simulink model "UPS_Vienna_TNPC"  (R2023b)
settings: Solver=ode45  StartTime=0.0  StopTime=0.5  RelTol=1e-3  EnableMultiTasking=on
libraries: spsSeriesRLCBranchLib x6, spsMosfetLib x6, spsCurrentMeasurementLib x4, spsVoltageMeasurementLib x4, spsDiodeLib x4, simulink x3, powerlib_extras x2, spsIGBTDiodeLib x2, spsTHDLib x2, spsACVoltageSourceLib x1, spsMeanLib x1, slpidlib x1
settings Model: SimulationMode=accelerator  Creator=bzz  LastModifiedBy=Qu
settings SolverCC: ZeroCrossAlgorithm=Adaptive  AlgebraicLoopSolver=TrustRegion
settings DataIOCC: LimitDataPoints=on  ReturnWorkspaceOutputs=off
settings OptimizationCC: LifeSpan=inf
settings DebuggingCC: AlgebraicLoopMsg=none  IgnoredZcDiagnostic=none  UnconnectedInputMsg=warning  UnconnectedOutputMsg=warning  UnconnectedLineMsg=warning  AllowSymbolicDim=off  SFUnexpectedBacktrackingDiag=warning  SFNoUnconditionalDefaultTransitionDiag=warning  ArithmeticOperatorsInVariantConditions=warning
settings ModelReferenceCC: EnableRefExpFcnMdlSchedulingChecks=on  PropagateSignalLabelsOutOfModel=off
settings SFSimCC: SimUseLocalCustomCode=off  CustomCodeUndefinedFunction=UseInterfaceOnly
settings RTWCC: RTWUseLocalCustomCode=off  DLArmComputeVersion=19.05
settings CodeAppCC: StateflowObjectComments=on
settings GRTTargetCC: TargetLangStandard=C89/C90 (ANSI)
settings ConfigComp: CovMetricSettings=dw  CovSaveCumulativeToWorkspaceVar=on  CovSaveSingleToWorkspaceVar=on  CovExternalEMLEnable=off
settings SimscapeCC: SimscapeNormalizeSystem=off

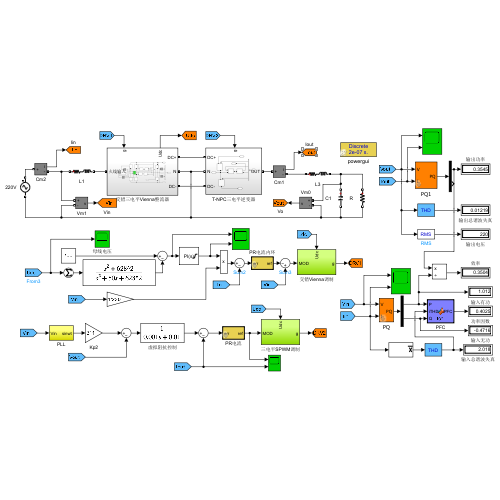
[thumbnail: Simulink's stored preview of the top-level diagram]
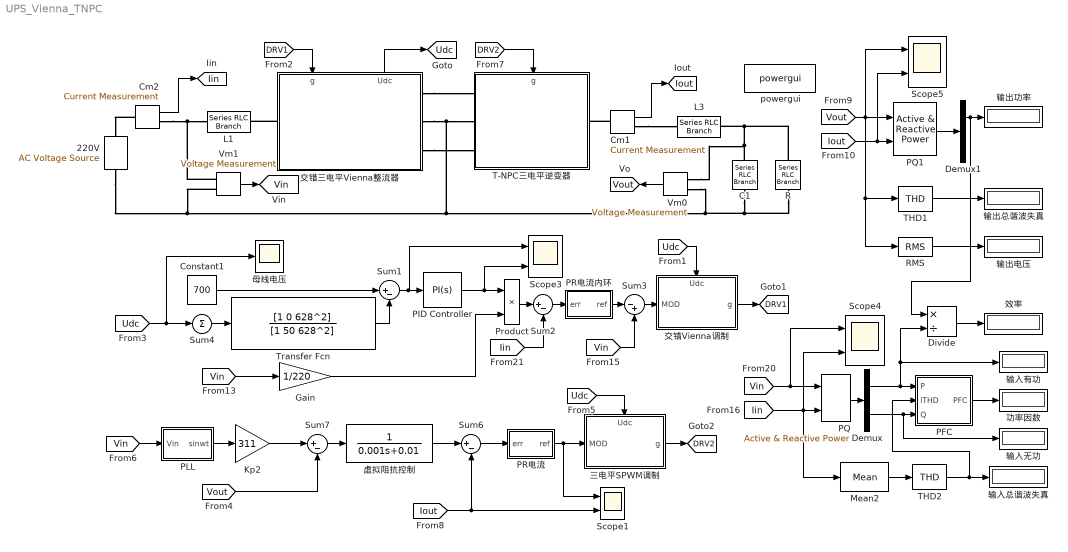
== system UPS_Vienna_TNPC ==
  220V : spsACVoltageSourceLib/AC Voltage Source  Amplitude=225*1.4  Phase=0  Frequency=50  SampleTime=0  Measurements=None  BusType=swing  Pref=10e3  Qref=0  Qmin=-inf  Qmax=+inf
  C1 : spsSeriesRLCBranchLib/Series RLC Branch  LConnTagsString=__new0  RConnTagsString=__new0  BranchType=C  Resistance=0.1  Inductance=0  SetiL0=off  InitialCurrent=0  Capacitance=6e-6  Setx0=off  InitialVoltage=310  Measurements=None
  Cm1 : spsCurrentMeasurementLib/Current Measurement  PhasorSimulation=off  OutputType=Complex  PSBequivalent=0
  Cm2 : spsCurrentMeasurementLib/Current Measurement  PhasorSimulation=off  OutputType=Complex  PSBequivalent=0
  Constant1 : Constant  Value=700
  Demux : Demux  Outputs=2
  Demux1 : Demux  Outputs=2
  Divide : Product  Inputs=*/
  Gain : Gain  Gain=1/220
  Kp2 : Gain  Gain=311
  L1 : spsSeriesRLCBranchLib/Series RLC Branch  LConnTagsString=__new0  RConnTagsString=__new0  BranchType=RL  Resistance=0.01  Inductance=3e-4  SetiL0=off  InitialCurrent=0  Capacitance=inf  Setx0=off  InitialVoltage=0  Measurements=None
  L3 : spsSeriesRLCBranchLib/Series RLC Branch  LConnTagsString=__new0  RConnTagsString=__new0  BranchType=RL  Resistance=0.01  Inductance=6e-4  SetiL0=off  InitialCurrent=0  Capacitance=inf  Setx0=off  InitialVoltage=0  Measurements=None
  Mean2 : spsMeanLib/Mean  Freq=10000  Vinit=0  Ts=0
  PFC : MATLAB Function  TreatAsAtomicUnit=on
  PID Controller : slpidlib/PID Controller  Controller=PI  Form=Parallel  TimeDomain=Continuous-time  UseExternalTs=off  SampleTime=-1  IntegratorMethod=Forward Euler  FilterMethod=Forward Euler  ControllerParametersSource=internal  P=0.2  I=4  UseKiTs=off  D=0.001  N=100  UseFilter=on  TunerSelectOption=Transfer Function Based (PID Tuner App)  InitialConditionSource=internal  InitialConditionForIntegrator=0  InitialConditionForFilter=0  DifferentiatorICPrevScaledInput=0  ExternalReset=none  TrackingMode=off  Kt=1  LimitOutput=on  SatLimitsSource=internal  UpperSaturationLimit=200  LowerSaturationLimit=-200  LinearizeAsGain=on  AntiWindupMode=clamping  Kb=1  LimitIntegrator=off  UpperIntegratorSaturationLimit=inf  LowerIntegratorSaturationLimit=-inf  POutMin=[]  POutMax=[]  IOutMin=[]  IOutMax=[]  DOutMin=[]  DOutMax=[]  NOutMin=[]  NOutMax=[]  SumOutMin=[]  SumOutMax=[]  SaturationOutMin=[]  SaturationOutMax=[]  PParamMin=[]  PParamMax=[]  IParamMin=[]  IParamMax=[]  DParamMin=[]  DParamMax=[]  NParamMin=[]  NParamMax=[]  KbParamMin=[]  KbParamMax=[]  KtParamMin=[]  KtParamMax=[]  KbOutMin=[]  KbOutMax=[]  KtOutMin=[]  KtOutMax=[]  IntegratorOutMin=[]  IntegratorOutMax=[]  FilterOutMin=[]  FilterOutMax=[]  SumI1OutMin=[]  SumI1OutMax=[]  SumI2OutMin=[]  SumI2OutMax=[]  SumI3OutMin=[]  SumI3OutMax=[]  SumI4OutMin=[]  SumI4OutMax=[]  SumDOutMin=[]  SumDOutMax=[]  DifferentiatorOutMin=[]  DifferentiatorOutMax=[]  FilterDiffOutCoefMin=[]  FilterDiffOutCoefMax=[]  ReciprocalOutMin=[]  ReciprocalOutMax=[]  SumDenOutMin=[]  SumDenOutMax=[]  SumNumOutMin=[]  SumNumOutMax=[]  DivideOutMin=[]  DivideOutMax=[]  UdiffTsProdOutMin=[]  UdiffTsProdOutMax=[]  NTsProdOutMin=[]  NTsProdOutMax=[]  UintegralTsProdOutMin=[]  UintegralTsProdOutMax=[]  UngainTsProdOutMin=[]  UngainTsProdOutMax=[]  ClampingZeroOutDataTypeStr=Inherit: Inherit via back propagation  ClampingZeroOutMin=[]  ClampingZeroOutMax=[]  FilterDenConstantOutDataTypeStr=Inherit: Inherit via back propagation  FilterDenConstantOutMin=[]  FilterDenConstantOutMax=[]  PCopyOutDataTypeStr=Inherit: Inherit via back propagation  PCopyOutMin=[]  PCopyOutMax=[]  NCopyOutDataTypeStr=Inherit: Inherit via back propagation  NCopyOutMin=[]  NCopyOutMax=[]  IntegratorContinuousStateAttributes=''  IntegratorStateMustResolveToSignalObject=off  IntegratorRTWStateStorageClass=Auto  FilterContinuousStateAttributes=''  FilterStateMustResolveToSignalObject=off  FilterRTWStateStorageClass=Auto  ParallelPVariant=InternalParameters  IdealPVariant=Disabled  IVariant=InternalParameters  DVariant=Disabled  IntegratorVariant=Continuous  SatVariant=Enabled  AWVariant=ContClampingParallel  PCopyVariant=Disabled  TRVariant=Disabled  FdbkBlocksVariant=Forward  IdealPFdbkVariant=Disabled  SatFdbkVariant=Disabled  DerivativeFilterVariant=Disabled  NVariant=Disabled  NCopyVariant=Disabled_SignalSpec  FilterICVariant=Disabled  IntegratorICVariant=InternalICs  ExternalResetVariant=Disabled  TRSumVariant=Passthrough  SumFdbkVariant=Disabled  SumVariant=Sum_PI  TsampFilterVariant=InternalTs  TsampNgainVariant=Passthrough  TsampIntegralVariant=Disabled_SignalSpec  ExternalSaturationOutDataTypeStr=Inherit: Same as second input
  PLL : Subsystem
  PQ : powerlib_extras/Measurements/Active & Reactive Power  f1=50
  PQ1 : powerlib_extras/Measurements/Active & Reactive Power  f1=50
  PR电流 : Subsystem  TreatAsAtomicUnit=on  mask{Kp=2, Kr=300, Wc=5, Upper=1000, Lower=-1000}
  PR电流内环 : Subsystem  TreatAsAtomicUnit=on  mask{Kp=6, Kr=100, Wc=5, Upper=310, Lower=-310}
  Product : Product
  R : spsSeriesRLCBranchLib/Series RLC Branch  LConnTagsString=__new0  RConnTagsString=__new0  BranchType=R  Resistance=15  Inductance=0  SetiL0=off  InitialCurrent=0  Capacitance=1e-5  Setx0=off  InitialVoltage=310  Measurements=None
  RMS : spsRMSLib/RMS  TrueRMS=on  Freq=50  RMSInit=200  Ts=0
  Scope{1,3..5} (4 alike) : Scope  NumInputPorts=2
  Sum{1..2,6..7} (4 alike) : Sum  Inputs=|+-
  Sum3 : Sum  Inputs=|-+
  Sum4 : Sum  Inputs=+
  T-NPC三电平逆变器 : Subsystem
      settings: PortSchema="{\"entries\":[{\"content\":{\"sides\":[{\"content\":{\"connectorIds\":[\"LConn1\",\"LConn2\",\"LConn3\"]},\"type\":\"ConnectorPlacement.EquallySpacedRectSide\",\"uuid\":\"7489be24-fb05-4397-99c4-0805e15884ae\"},{\"content\":{\"connectorIds\":[\"RConn1\"],\"side\":\"RIGHT\"},\"type\":\"ConnectorPlacement.EquallySpacedRectSide\",\"uuid\":\"654e1801-31b1-421a-885f-2131c51cad8d\"},{\"content\":{\"connectorIds\":[\"In1\"],\"side\":\"TOP\"},\"type\":\"ConnectorPlacement.EquallySpacedRectSide\",\"uuid\":\"fb480e4b-a2b2-44a5-99b2-e83f2782ffff\"},{\"content\":{\"side\":\"BOTTOM\"},\"type\":\"ConnectorPlacement.EquallySpacedRectSide\",\"uuid\":\"4af6c17e-9b76-400a-bd3e-3ab3838d4ab0\"}]},\"type\":\"ConnectorPlacement.EquallySpacedConnector\",\"uuid\":\"da460d4a-b9c7-40d8-ac01-f49018117654\"}],\"packageUris\":[\"http://schema.mathworks.com/mf0/Connector/R2020b\"],\"version\":\"1.0\"}"
  THD1 : spsTHDLib/THD  Freq=50  Ts=0
  THD2 : spsTHDLib/THD  Freq=50  Ts=0
  Transfer Fcn : TransferFcn  Numerator=[1 0 628^2]  Denominator=[1 50 628^2]
  Vm0 : spsVoltageMeasurementLib/Voltage Measurement  PhasorSimulation=off  OutputType=Complex  PSBequivalent=0
  Vm1 : spsVoltageMeasurementLib/Voltage Measurement  PhasorSimulation=off  OutputType=Complex  PSBequivalent=0
  powergui : spspowerguiLib/powergui  SimulationMode=Discrete  SampleTime=2e-7  frequency=60  Iterations=50  frequencyindice=0  Pbase=100e6  ErrMax=1e-4  UnitsV=kV  UnitsW=MW  buscounter=0  FunctionMessages=off  echomessages=off  EnableUseOfTLC=off  CurrentSourceSwitches=off  DisableSnubberDevices=off  DisableRonSwitches=off  DisableVfSwitches=off  DisplayEquations=off  AutomaticDiscreteSolvers=off  SolverType=Tustin/Backward Euler (TBE)  Interpol=off  ExternalGateDelay=off  methode=off  Ts=0  x0status=blocks  SPID=off  SwTol=0  HookPort=off  NonlinearTolerance=1e-4  nMaxIteration=100  ContinueOnMaxIteration=off  RestoreLinks=warning  ResistiveCurrentMeasurement=off  Frange=[0:2:500]  Ylog=off  Xlog=on  ShowGrid=off  save=off  variable=ZData  structure=QQQQQ  ZoomFFT=off  StartTime=0.5  cycles=15  DisplayStyle=1  fundamental=50  FreqAxis=off  MaxFrequency=1000  frequencyindicesteady=1  RmsSteady=1  display=off
  三电平SPWM调制 : Subsystem
      settings: PortSchema="{\"entries\":[{\"content\":{\"sides\":[{\"content\":{\"connectorIds\":[\"In1\"]},\"type\":\"ConnectorPlacement.EquallySpacedRectSide\",\"uuid\":\"1b638a2d-5755-4ae9-be2e-6e83381e6ec7\"},{\"content\":{\"connectorIds\":[\"Out1\"],\"side\":\"RIGHT\"},\"type\":\"ConnectorPlacement.EquallySpacedRectSide\",\"uuid\":\"c11d6821-83ca-44ae-8b26-9c21f079c52d\"},{\"content\":{\"connectorIds\":[\"In2\"],\"side\":\"TOP\"},\"type\":\"ConnectorPlacement.EquallySpacedRectSide\",\"uuid\":\"290bd415-8c82-45df-a08c-f8079695ccf4\"}]},\"type\":\"ConnectorPlacement.EquallySpacedConnector\",\"uuid\":\"c88eaf66-3c08-44e5-8886-a76105e28a39\"}],\"packageUris\":[\"http://schema.mathworks.com/mf0/Connector/R2020b\"],\"version\":\"1.0\"}"
  交错Vienna调制 : Subsystem
      settings: PortSchema="{\"entries\":[{\"content\":{\"sides\":[{\"content\":{\"connectorIds\":[\"In1\"]},\"type\":\"ConnectorPlacement.EquallySpacedRectSide\",\"uuid\":\"1b638a2d-5755-4ae9-be2e-6e83381e6ec7\"},{\"content\":{\"connectorIds\":[\"Out1\"],\"side\":\"RIGHT\"},\"type\":\"ConnectorPlacement.EquallySpacedRectSide\",\"uuid\":\"c11d6821-83ca-44ae-8b26-9c21f079c52d\"},{\"content\":{\"connectorIds\":[\"In2\"],\"side\":\"TOP\"},\"type\":\"ConnectorPlacement.EquallySpacedRectSide\",\"uuid\":\"290bd415-8c82-45df-a08c-f8079695ccf4\"}]},\"type\":\"ConnectorPlacement.EquallySpacedConnector\",\"uuid\":\"c88eaf66-3c08-44e5-8886-a76105e28a39\"}],\"packageUris\":[\"http://schema.mathworks.com/mf0/Connector/R2020b\"],\"version\":\"1.0\"}"
  交错三电平Vienna整流器 : Subsystem
      settings: PortSchema="{\"entries\":[{\"content\":{\"sides\":[{\"content\":{\"connectorIds\":[\"LConn1\"]},\"type\":\"ConnectorPlacement.EquallySpacedRectSide\",\"uuid\":\"7489be24-fb05-4397-99c4-0805e15884ae\"},{\"content\":{\"connectorIds\":[\"RConn1\",\"RConn2\",\"RConn3\"],\"side\":\"RIGHT\"},\"type\":\"ConnectorPlacement.EquallySpacedRectSide\",\"uuid\":\"654e1801-31b1-421a-885f-2131c51cad8d\"},{\"content\":{\"connectorIds\":[\"In1\",\"Out1\"],\"side\":\"TOP\"},\"type\":\"ConnectorPlacement.EquallySpacedRectSide\",\"uuid\":\"fb480e4b-a2b2-44a5-99b2-e83f2782ffff\"},{\"content\":{\"side\":\"BOTTOM\"},\"type\":\"ConnectorPlacement.EquallySpacedRectSide\",\"uuid\":\"4af6c17e-9b76-400a-bd3e-3ab3838d4ab0\"}]},\"type\":\"ConnectorPlacement.EquallySpacedConnector\",\"uuid\":\"da460d4a-b9c7-40d8-ac01-f49018117654\"}],\"packageUris\":[\"http://schema.mathworks.com/mf0/Connector/R2020b\"],\"version\":\"1.0\"}"
  功率因数 : Display
  效率 : Display
  母线电压 : Scope
  虚拟阻抗控制 : TransferFcn  Numerator=1  Denominator=[0.001 0.01]
  输入总谐波失真 : Display
  输入无功 : Display
  输入有功 : Display
  输出功率 : Display
  输出总谐波失真 : Display
  输出电压 : Display
  tag scope: DRV1=global, DRV2=global, Iin=global, Iout=global, Udc=global, Vin=global, Vout=global
  wires:
  PQ/1 -> Demux/1
  Demux/2 -> 输入无功/1, PFC/3(Q)
  PFC/1(PFC) -> 功率因数/1
  Demux/1 -> Divide/2, 输入有功/1, PFC/1(P)
  Cm1/1 -> [Iout]
  THD1/1 -> 输出总谐波失真/1
  Sum1/1 -> Scope3/1, PID Controller/1
  [Vin] -> PQ/1, Scope4/1
  Mean2/1 -> THD2/1
  THD2/1 -> 输入总谐波失真/1, PFC/2(iTHD)
  PR电流内环/1(ref) -> Sum3/1
  [Iin] -> Sum2/2
  Sum2/1 -> PR电流内环/1(err)
  Product/1 -> Sum2/1
  PID Controller/1 -> Product/1, Scope3/2
  交错Vienna调制/1(g) -> [DRV1]
  Constant1/1 -> Sum1/1
  [Udc] -> 母线电压/1, Sum4/1
  Sum4/1 -> Transfer Fcn/1
  Transfer Fcn/1 -> Sum1/2
  [Iin] -> Mean2/1, Scope4/2, PQ/2
  [Vin] -> Gain/1
  Sum3/1 -> 交错Vienna调制/1(MOD)
  [Udc] -> 交错Vienna调制/2(Udc)
  [Vin] -> Sum3/2
  交错三电平Vienna整流器/1(Udc) -> [Udc]
  [Iout] -> Scope1/2, Sum6/2
  Sum7/1 -> 虚拟阻抗控制/1
  PLL/1(sinwt) -> Kp2/1
  Kp2/1 -> Sum7/1
  [Vin] -> PLL/1(Vin)
  [Vout] -> Sum7/2
  虚拟阻抗控制/1 -> Sum6/1
  Sum6/1 -> PR电流/1(err)
  三电平SPWM调制/1(g) -> [DRV2]
  [Udc] -> 三电平SPWM调制/2(Udc)
  [DRV2] -> T-NPC三电平逆变器/1(g)
  Vm0/1 -> [Vout]
  [DRV1] -> 交错三电平Vienna整流器/1(g)
  Gain/1 -> Product/2
  Vm1/1 -> [Vin]
  Cm2/1 -> [Iin]
  PR电流/1(ref) -> Scope1/1, 三电平SPWM调制/1(MOD)
  RMS/1 -> 输出电压/1
  [Vout] -> Scope5/1, RMS/1, THD1/1, PQ1/1
  [Iout] -> Scope5/2, PQ1/2
  PQ1/1 -> Demux1/1
  Demux1/1 -> Divide/1, 输出功率/1
  Divide/1 -> 效率/1
  connections:
  Cm1/RConn1 -- L3/LConn1
  交错三电平Vienna整流器/LConn1 -- L1/RConn1
  220V/LConn1 -- Vm1/LConn2 -- R/RConn1 -- C1/RConn1 -- Vm0/LConn2 -- T-NPC三电平逆变器/LConn2 -- 交错三电平Vienna整流器/RConn2
  Cm1/LConn1 -- T-NPC三电平逆变器/RConn1
  C1/LConn1 -- L3/RConn1 -- R/LConn1 -- Vm0/LConn1
  交错三电平Vienna整流器/RConn1 -- T-NPC三电平逆变器/LConn1
  交错三电平Vienna整流器/RConn3 -- T-NPC三电平逆变器/LConn3
  Cm2/LConn1 -- 220V/RConn1
  Cm2/RConn1 -- Vm1/LConn1 -- L1/LConn1

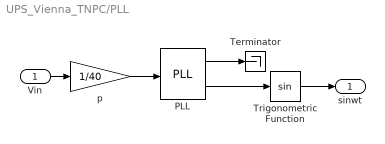
== system UPS_Vienna_TNPC/PLL ==
  Vin : Inport
  PLL : spsPLLLib/PLL  Fmin=45  Par_Init=[0, 50]  ParK=[180, 3200, 1]  TcD=1e-4  MaxRateChangeFreq=12  FilterCutOffFreq=25  Ts=0  AGC=on
  Terminator : Terminator
  Trigonometric Function : Trigonometry
  p : Gain  Gain=1/40
  sinwt : Outport
  wires:
  PLL/2 -> Trigonometric Function/1
  PLL/1 -> Terminator/1
  p/1 -> PLL/1
  Trigonometric Function/1 -> sinwt/1
  Vin/1 -> p/1

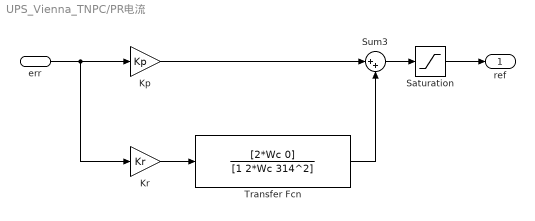
== system UPS_Vienna_TNPC/PR电流 ==
  err : Inport
  Kp : Gain  Gain=Kp
  Kr : Gain  Gain=Kr
  Saturation : Saturate  UpperLimit=Upper  LowerLimit=Lower
  Sum3 : Sum  Inputs=|++
  Transfer Fcn : TransferFcn  Numerator=[2*Wc 0]  Denominator=[1 2*Wc 314^2]
  ref : Outport
  wires:
  Kp/1 -> Sum3/1
  Sum3/1 -> Saturation/1
  err/1 -> Kr/1, Kp/1
  Kr/1 -> Transfer Fcn/1
  Transfer Fcn/1 -> Sum3/2
  Saturation/1 -> ref/1

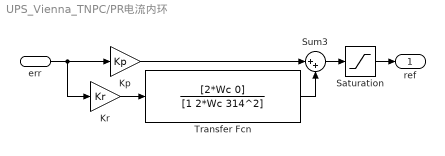
== system UPS_Vienna_TNPC/PR电流内环 ==
  err : Inport
  Kp : Gain  Gain=Kp
  Kr : Gain  Gain=Kr
  Saturation : Saturate  UpperLimit=Upper  LowerLimit=Lower
  Sum3 : Sum  Inputs=|++
  Transfer Fcn : TransferFcn  Numerator=[2*Wc 0]  Denominator=[1 2*Wc 314^2]
  ref : Outport
  wires:
  Kp/1 -> Sum3/1
  Kr/1 -> Transfer Fcn/1
  Transfer Fcn/1 -> Sum3/2
  Saturation/1 -> ref/1
  err/1 -> Kr/1, Kp/1
  Sum3/1 -> Saturation/1

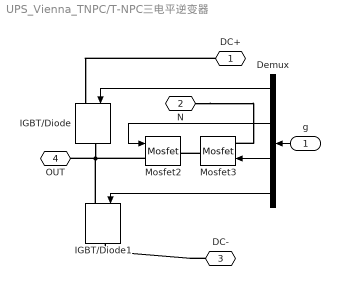
== system UPS_Vienna_TNPC/T-NPC三电平逆变器 ==
  g : Inport
  Demux : Demux
  IGBT/Diode : spsIGBTDiodeLib/IGBT//Diode  Ron=1e-2  Rs=1e5  Cs=inf  Measurements=off
  IGBT/Diode1 : spsIGBTDiodeLib/IGBT//Diode  Ron=1e-2  Rs=1e5  Cs=inf  Measurements=off
  Mosfet2 : spsMosfetLib/Mosfet  Ron=0.05  Lon=0  Rd=0.01  Vfd=1  IC=0  Rs=1e5  Cs=inf  Measurements=off
  Mosfet3 : spsMosfetLib/Mosfet  Ron=0.05  Lon=0  Rd=0.01  Vfd=1  IC=0  Rs=1e5  Cs=inf  Measurements=off
  DC+ : PMIOPort  Side=Left
  N : PMIOPort  Port=2  Side=Left
  DC- : PMIOPort  Port=3  Side=Left
  OUT : PMIOPort  Port=4  Side=Right
  wires:
  g/1 -> Demux/1
  Demux/3 -> Mosfet3/1
  Demux/2 -> Mosfet2/1
  Demux/1 -> IGBT/Diode/1
  Demux/4 -> IGBT/Diode1/1
  connections:
  Mosfet2/LConn1 -- IGBT/Diode1/LConn1 -- IGBT/Diode/RConn1 -- OUT/RConn1
  Mosfet3/RConn1 -- Mosfet2/RConn1
  DC+/RConn1 -- IGBT/Diode/LConn1
  DC-/RConn1 -- IGBT/Diode1/RConn1
  N/RConn1 -- Mosfet3/LConn1

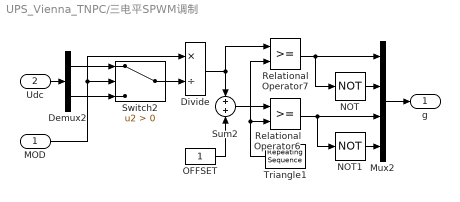
== system UPS_Vienna_TNPC/三电平SPWM调制 ==
  MOD : Inport
  Udc : Inport  Port=2
  Demux2 : Demux  Outputs=2
  Divide : Product  Inputs=*/
  Mux2 : Mux
  NOT : Logic  Operator=NOT  IconShape=distinctive  AllPortsSameDT=off  OutDataTypeStr=boolean
  NOT1 : Logic  Operator=NOT  IconShape=distinctive  AllPortsSameDT=off  OutDataTypeStr=boolean
  OFFSET : Constant
  Relational Operator6 : RelationalOperator  OutDataTypeStr=boolean  InputSameDT=off
  Relational Operator7 : RelationalOperator  OutDataTypeStr=boolean  InputSameDT=off
  Sum2 : Sum  Inputs=+|+
  Switch2 : Switch  Criteria=u2 > Threshold  SaturateOnIntegerOverflow=off  InputSameDT=off
  Triangle1 : simulink/Sources/Repeating Sequence  rep_seq_t=[0 1/33000/2 1/33000]  rep_seq_y=[0 1 0]
  g : Outport
  wires:
  Udc/1 -> Demux2/1
  MOD/1 -> Divide/1, Switch2/2
  Demux2/2 -> Switch2/3
  Switch2/1 -> Divide/2
  Demux2/1 -> Switch2/1
  Mux2/1 -> g/1
  Relational Operator7/1 -> NOT/1, Mux2/1
  OFFSET/1 -> Sum2/2
  Sum2/1 -> Relational Operator6/1
  Triangle1/1 -> Relational Operator7/2, Relational Operator6/2
  NOT/1 -> Mux2/2
  Relational Operator6/1 -> NOT1/1, Mux2/3
  NOT1/1 -> Mux2/4
  Divide/1 -> Relational Operator7/1, Sum2/1

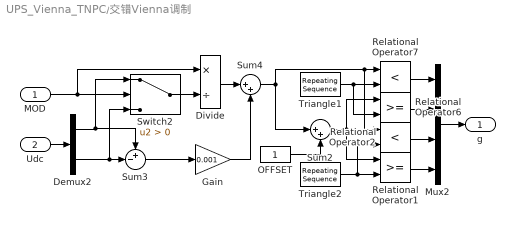
== system UPS_Vienna_TNPC/交错Vienna调制 ==
  MOD : Inport
  Udc : Inport  Port=2
  Demux2 : Demux  Outputs=2
  Divide : Product  Inputs=*/
  Gain : Gain  Gain=0.001
  Mux2 : Mux
  OFFSET : Constant
  Relational Operator1 : RelationalOperator  OutDataTypeStr=boolean  InputSameDT=off
  Relational Operator2 : RelationalOperator  Operator=<  OutDataTypeStr=boolean  InputSameDT=off
  Relational Operator6 : RelationalOperator  OutDataTypeStr=boolean  InputSameDT=off
  Relational Operator7 : RelationalOperator  Operator=<  OutDataTypeStr=boolean  InputSameDT=off
  Sum2 : Sum  Inputs=|++
  Sum3 : Sum  Inputs=+-|
  Sum4 : Sum  Inputs=|++
  Switch2 : Switch  Criteria=u2 > Threshold  SaturateOnIntegerOverflow=off  InputSameDT=off
  Triangle1 : simulink/Sources/Repeating Sequence  rep_seq_t=[0 1/33000/2 1/33000]  rep_seq_y=[0 1 0]
  Triangle2 : simulink/Sources/Repeating Sequence  rep_seq_t=[0 1/33000/2 1/33000]  rep_seq_y=[1 0 1]
  g : Outport
  wires:
  Triangle1/1 -> Relational Operator7/2, Relational Operator6/2
  Relational Operator6/1 -> Mux2/2
  Relational Operator7/1 -> Mux2/1
  OFFSET/1 -> Sum2/2
  Sum2/1 -> Relational Operator1/1, Relational Operator6/1
  Mux2/1 -> g/1
  Switch2/1 -> Divide/2
  Demux2/2 -> Switch2/3, Sum3/2
  MOD/1 -> Divide/1, Switch2/2
  Udc/1 -> Demux2/1
  Sum3/1 -> Gain/1
  Sum4/1 -> Sum2/1, Relational Operator2/1, Relational Operator7/1
  Divide/1 -> Sum4/1
  Gain/1 -> Sum4/2
  Demux2/1 -> Switch2/1, Sum3/1
  Relational Operator1/1 -> Mux2/4
  Relational Operator2/1 -> Mux2/3
  Triangle2/1 -> Relational Operator2/2, Relational Operator1/2

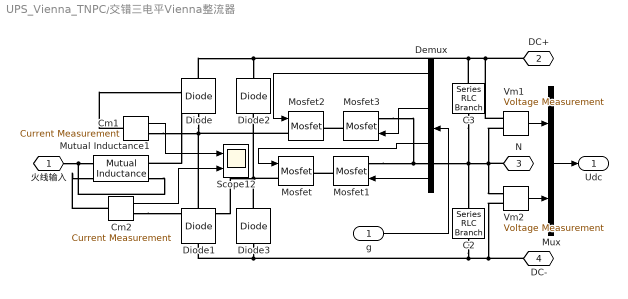
== system UPS_Vienna_TNPC/交错三电平Vienna整流器 ==
  g : Inport
  C2 : spsSeriesRLCBranchLib/Series RLC Branch  LConnTagsString=__new0  RConnTagsString=__new0  BranchType=C  Resistance=0.1  Inductance=0  SetiL0=off  InitialCurrent=0  Capacitance=4e-3  Setx0=on  InitialVoltage=310  Measurements=None
  C3 : spsSeriesRLCBranchLib/Series RLC Branch  LConnTagsString=__new0  RConnTagsString=__new0  BranchType=C  Resistance=0.1  Inductance=0  SetiL0=off  InitialCurrent=0  Capacitance=4e-3  Setx0=on  InitialVoltage=310  Measurements=None
  Cm1 : spsCurrentMeasurementLib/Current Measurement  PhasorSimulation=off  OutputType=Complex  PSBequivalent=0
  Cm2 : spsCurrentMeasurementLib/Current Measurement  PhasorSimulation=off  OutputType=Complex  PSBequivalent=0
  Demux : Demux
  Diode{,1..3} (4 alike) : spsDiodeLib/Diode  Ron=0.001  Lon=0  Vf=1  IC=0  UseSnubber=0  Rs=47  Cs=1e-9  Measurements=off
  Mosfet{,1..3} (4 alike) : spsMosfetLib/Mosfet  Ron=0.05  Lon=0  Rd=0.01  Vfd=1  IC=0  Rs=1e5  Cs=inf  Measurements=off
  Mutual Inductance1 : spsMutualInductanceLib/Mutual Inductance  LConnTagsString=a|b  RConnTagsString=A|B  TypeOfMutual=Two or three windings with equal mutual terms  NumberOfWindings=3  SelfImpedance1=[0.01 2e-3]  SelfImpedance2=[0.01 2e-3]  ThreeWindings=off  SelfImpedance3=[ 1.1 1.1e-03]  MutualImpedance=[0.02 1.95e-4]  InductanceMatrix="[1.0 0.9  0.9 ;  0.9 1.0  0.9;  0.9 0.9 1.0 ] * 1e-3"  ResistanceMatrix="[1.0 0.9  0.9 ;  0.9 1.0  0.9;  0.9 0.9 1.0 ]"  Measurements=None
  Mux : Mux  Inputs=2
  Scope12 : Scope  NumInputPorts=2
  Vm1 : spsVoltageMeasurementLib/Voltage Measurement  PhasorSimulation=off  OutputType=Complex  PSBequivalent=0
  Vm2 : spsVoltageMeasurementLib/Voltage Measurement  PhasorSimulation=off  OutputType=Complex  PSBequivalent=0
  火线输入 : PMIOPort  Side=Left
  DC+ : PMIOPort  Port=2  Side=Right
  N : PMIOPort  Port=3  Side=Right
  DC- : PMIOPort  Port=4  Side=Right
  Udc : Outport
  wires:
  Demux/4 -> Mosfet1/1
  Demux/3 -> Mosfet/1
  Demux/2 -> Mosfet3/1
  Demux/1 -> Mosfet2/1
  g/1 -> Demux/1
  Mux/1 -> Udc/1
  Vm1/1 -> Mux/1
  Vm2/1 -> Mux/2
  Cm1/1 -> Scope12/1
  Cm2/1 -> Scope12/2
  connections:
  Mosfet3/RConn1 -- Mosfet2/RConn1
  Mosfet1/RConn1 -- Mosfet/RConn1
  DC-/RConn1 -- C2/RConn1 -- Diode3/LConn1 -- Diode1/LConn1 -- Vm2/LConn2
  Diode/LConn1 -- Cm1/RConn1 -- Diode1/RConn1 -- Mosfet2/LConn1
  Diode/RConn1 -- C3/LConn1 -- Vm1/LConn1 -- DC+/RConn1 -- Diode2/RConn1
  Diode2/LConn1 -- Diode3/RConn1 -- Cm2/RConn1 -- Mosfet/LConn1
  Mosfet3/LConn1 -- Mosfet1/LConn1 -- C3/RConn1 -- N/RConn1 -- Vm2/LConn1 -- Vm1/LConn2 -- C2/LConn1
  火线输入/RConn1 -- Mutual Inductance1/RConn2 -- Mutual Inductance1/LConn1
  Cm2/LConn1 -- Mutual Inductance1/LConn2
  Cm1/LConn1 -- Mutual Inductance1/RConn1

== matlab function UPS_Vienna_TNPC/PFC ==
  data: P input; iTHD input; PFC output; Q input
function PFC = fcn(P,iTHD,Q)
% This block supports an embeddable subset of the MATLAB language.
% See the help menu for details. 
PFC=(P/sqrt(P*P+Q*Q))/sqrt(1+iTHD*iTHD);
